simulink model "demoPassiveWavefilterAutopilot2"  (R2022a)
settings: Solver=ode4  StartTime=0.0  StopTime=200  FixedStep=0.1  RelTol=1e-3  EnableMultiTasking=on
libraries: simulink_extras x5, simulink x2, mssSimulink x2
settings Model: Creator=thor  LastModifiedBy=thor
settings SolverCC: AlgebraicLoopSolver=TrustRegion
settings DataIOCC: LimitDataPoints=on  SaveFormat=Array  SignalLoggingSaveFormat=ModelDataLogs  ReturnWorkspaceOutputs=off  SignalLoggingName=sigsOut
settings OptimizationCC: BooleanDataType=off  InitFltsAndDblsToZero=on  LifeSpan=inf
settings DebuggingCC: SaveWithParameterizedLinksMsg=none  UnderspecifiedInitializationDetection=Classic  MergeDetectMultiDrivingBlocksExec=none  SignalResolutionControl=TryResolveAllWithWarning  MultiTaskDSMMsg=warning  MultiTaskCondExecSysMsg=none  FcnCallInpInsideContextMsg=warning  UnconnectedInputMsg=warning  UnconnectedOutputMsg=warning  UnconnectedLineMsg=warning  SFUnexpectedBacktrackingDiag=warning  SFNoUnconditionalDefaultTransitionDiag=warning  SFExecutionAtInitializationDiag=none  SFMachineParentedDataDiag=warning  ArithmeticOperatorsInVariantConditions=warning
settings HardwareCC: ProdBitPerPointer=32  ProdBitPerSizeT=32  ProdBitPerPtrDiffT=32  ProdLargestAtomicFloat=None  ProdIntDivRoundTo=Undefined  ProdEndianess=Unspecified  ProdWordSize=32  ProdHWDeviceType=32-bit Generic  TargetUnknown=on
settings ModelReferenceCC: PropagateSignalLabelsOutOfModel=off
settings RTWCC: DLArmComputeVersion=19.05
settings CodeAppCC: StateflowObjectComments=on
settings GRTTargetCC: TargetFcnLib=ansi_tfl_tmw.mat  TargetLangStandard=C89/C90 (ANSI)  ModelReferenceCompliant=off  CombineOutputUpdateFcns=off  MatFileLogging=off  GRTInterface=on
settings ConfigComp: CovMetricSettings=dw  CovSaveCumulativeToWorkspaceVar=on  CovSaveSingleToWorkspaceVar=on

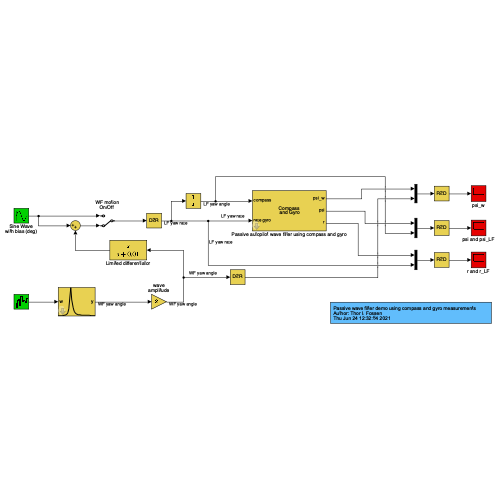
[thumbnail: Simulink's stored preview of the top-level diagram]
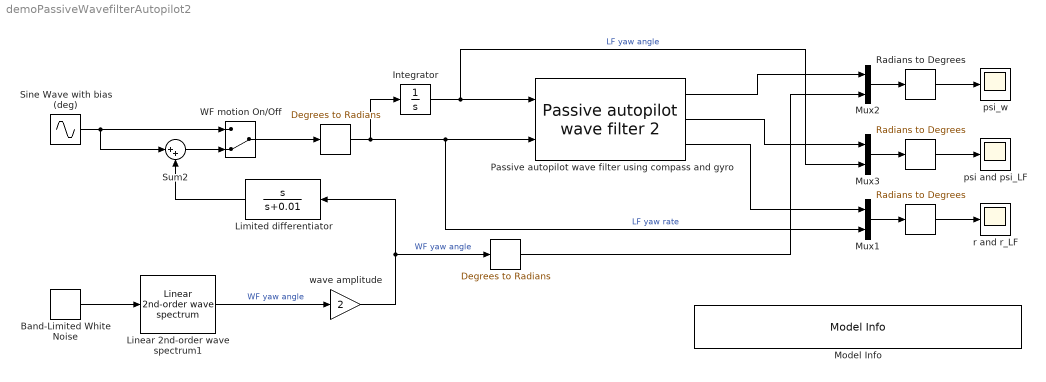
== system demoPassiveWavefilterAutopilot2 ==
  " " : simulink_extras/Transformations/Radians to Degrees
  "  " : simulink_extras/Transformations/Radians to Degrees
  "   " : simulink_extras/Transformations/Degrees to Radians
  "        " : simulink_extras/Transformations/Degrees to Radians
  Band-Limited White Noise : simulink/Sources/Band-Limited White Noise  Cov=[1]  Ts=0.1  seed=[23341]
  Integrator : Integrator
  Limited differentiator : TransferFcn  Numerator=[1 0]  Denominator=[1 0.01]
  Linear 2nd-order wave spectrum1 : mssSimulink/Environment/Waves/Linear 2nd-order  wave spectrum  sigma=0.5  w_0=1.2  lambda=0.1
  Model Info : simulink/Model-Wide Utilities/Model Info  Frame=on  DisplayStringWithTags=|  HorizontalTextAlignment=Left  LeftAlignmentValue=0.02
      | Passive wave filter demo using compass and gyro measurements
      | Author: Thor I. Fossen
      | %<LastModificationDate>
  Mux1 : Mux  Inputs=2
  Mux2 : Mux  Inputs=2
  Mux3 : Mux  Inputs=2
  Passive autopilot wave filter using compass and gyro : mssSimulink/Navigation/Estimators/Passive autopilot wave filter 2  lambda=0.1  w_o=1.2  K4=0.1  zeta_n=0.01  w_c=2  T_b=100
  "Radians to Degrees  " : simulink_extras/Transformations/Radians to Degrees
  Sine Wave with bias (deg) : Sin  Amplitude=0.5  Frequency=0.1  SampleTime=0
  Sum2 : Sum  Inputs=|++  InputSameDT=on  SaturateOnIntegerOverflow=on  OutDataTypeStr=Inherit: Same as first input
  "WF motion On/Off " : ManualSwitch  CurrentSetting=0
  psi and psi_LF : Scope
  psi_w : Scope
  r and r_LF : Scope
  wave amplitude : Gain  Gain=2  SaturateOnIntegerOverflow=on  OutDataTypeStr=Inherit: Same as input  ParamDataTypeStr=Inherit: Same as input
  wires:
  Band-Limited White Noise/1 -> Linear 2nd-order wave spectrum1/1
  Mux2/1 -> "Radians to Degrees  "/1
  "Radians to Degrees  "/1 -> psi_w/1
  " "/1 -> psi and psi_LF/1
  Mux1/1 -> "  "/1
  "  "/1 -> r and r_LF/1
  "WF motion On/Off "/1 -> "        "/1
  Linear 2nd-order wave spectrum1/1 -> wave amplitude/1  "WF yaw angle"
  Passive autopilot wave filter using compass and gyro/3 -> Mux1/1
  Integrator/1 -> Passive autopilot wave filter using compass and gyro/1, Mux3/2  "LF yaw angle"
  Sine Wave with bias (deg)/1 -> "WF motion On/Off "/1, Sum2/1
  Sum2/1 -> "WF motion On/Off "/2
  "        "/1 -> Passive autopilot wave filter using compass and gyro/2, Mux1/2, Integrator/1  "LF yaw rate"
  Passive autopilot wave filter using compass and gyro/2 -> Mux3/1
  Mux3/1 -> " "/1
  wave amplitude/1 -> "   "/1, Limited differentiator/1  "WF yaw angle"
  Limited differentiator/1 -> Sum2/2
  Passive autopilot wave filter using compass and gyro/1 -> Mux2/1
  "   "/1 -> Mux2/2
